simulink model "launch_gate_exp"  (R2022b)
settings: Solver=FixedStepDiscrete  StartTime=0.0  StopTime=5  FixedStep=0.001  RelTol=1e-3
InitFcn:
  | if ~exist('P','var') || ~isfield(P,'gate_version'), P=gate_params(launch_tcs_params()); end
model workspace (MAT data in the model file):
  w_2 : Simulink.Parameter (value not decoded)
undefined symbols (not defined in the file): A, a, B, b, C, D, DiscIntNeverNeededParam, Iz, K, k1, K1, k2, K2, L1, L2, m, magnitude, Phi, Sample_time, Steer_Ratio
libraries: simulink x26, slpidlib x13, Solver_SF x1, dsparch4 x1
(part 7 of 7)

== matlab function launch_gate_exp/PID_Controller//直线循迹/MATLAB Function2 ==
  data: st input; flag_ctrl output; flag_cnt output; yaw input; throttle input; yaw_ref output
function [flag_ctrl, flag_cnt, yaw_ref] = StraightModeDetector(st, yaw, throttle)

%% 实车调试版本
% 所有 persistent 变量必须为 single 以满足实车要求 
persistent ctrl_cnt yaw_sum yaw_time yaw_ref_int yaw_f
if isempty(ctrl_cnt)
    ctrl_cnt    = single(0);
    yaw_sum     = single(0);
    yaw_time    = single(0);
    yaw_ref_int = single(0);
    yaw_f       = single(0);
end

%% === 参数 ===
st_lim_enter = single(1);     % 进入判定阈值 (deg)
st_lim_exit  = single(1.2);     % 退出判定（滞回）
thr_min      = single(1);       % 油门下限 (%)
thr_max      = single(50);      % 油门上限 (%)


T_ctrl   = single(3.0);         % 需要检测的直行时间 (s)
Ts       = single(0.02);        % sample time
num_ctrl = single(T_ctrl / Ts); % 循环次数

alpha = single(0.15);           % LPF 低通滤波器系数
flag_cnt = single(0);           % 累加计算目标航向使能

%% === Step 1: LPF 过滤 yaw ===
yaw_f = yaw_f + alpha * (yaw - yaw_f);

%% === Step 2: 判断是否满足直行条件 ===
cond_enter = (abs(st) < st_lim_enter) && (throttle > thr_min) && (throttle < thr_max);
cond_exit  = (abs(st) > st_lim_exit)  || (throttle <= thr_min) || (throttle >= thr_max);

%% === Step 3: 计数器逻辑 ===
if cond_enter
    ctrl_cnt = ctrl_cnt + 1;
else
    ctrl_cnt = single(0);
end

%% === Step 4: yaw 采样（累加）===
if cond_enter && (ctrl_cnt <= num_ctrl)
    yaw_sum  = yaw_sum  + yaw_f;
    yaw_time = yaw_time + 1;
    flag_cnt = single(1);
end

%% === Step 5: 进入直线控制模式的瞬间冻结 yaw_ref ===
% if ctrl_cnt == num_ctrl
%     yaw_ref_int = yaw_sum / yaw_time;
% end
if (ctrl_cnt >= num_ctrl) && (yaw_time > 0) && (yaw_ref_int == 0)
    yaw_ref_int = yaw_sum / yaw_time;
end

%% === Step 6: 若退出模式，则清空状态 ===
if cond_exit
    ctrl_cnt    = single(0);
    yaw_sum     = single(0);
    yaw_time    = single(0);
    yaw_ref_int = single(0);
end

%% === Step 7: 输出 ===
flag_ctrl = single(ctrl_cnt >= num_ctrl);
yaw_ref   = yaw_ref_int;

end

== matlab function launch_gate_exp/PID_Controller//直线循迹/指数加权移动平均 ==
  data: uk input; y output; is_biased input

function y = ExpMovAvg(uk, is_biased)
% 指数加权移动平均滤波器
% 输入:
%   uk      : 当前输入值
%   is_biased: 是否应用偏差修正 (1=是, 0=否)
% 输出:
%   y       : 指数加权移动平均值

% 持久变量保持状态 (在时间步之间保留值)
persistent shadow count first_time decay

% 初始化参数和状态
if isempty(first_time)
    % 初始化标志
    first_time = true;
    
    % 初始化状态值
    shadow = double(0);
    count = 0;
    
    % 设置衰减因子 (0.9是常用值，可根据需要修改)
    decay = 0.9;
end

% 主处理逻辑
if first_time
    % 第一次调用 - 初始化状态
    shadow = double(uk);
    count = 1;
    first_time = false;
    y = uk;  % 第一次返回当前值
else
    % 更新计数器
    count = count + 1;
    
    % 计算指数加权平均值
     a = decay * shadow + (1 - decay) * uk;
    shadow = double(a);
    
    if is_biased
        % 应用偏差修正 (1 - decay^count)
        bias_correction = 1 - decay^count;
         b = shadow / bias_correction;
        y = single(b);
    else
        % 返回原始加权平均值
        y = single(shadow);
    end
end
end

== matlab function launch_gate_exp/PID_Controller//直线循迹/模式判断 ==
  data: v input; st input; avg input; mode output
function mode  = stateflow(v,st,avg)

mode = 7; %常规模式

% 沥青路面判断
    if avg <= 2
        if v > 20
            if st>=8
                mode = 1; % 高速转向
            elseif st<=3
                mode = 2; % 高速直行
            end
        elseif v < 10
            if st>=5
                mode = 3; % 低速转向
            elseif st<5
                mode = 4; % 低速直行
            end
        end
    % 土地路面判断
    elseif avg >= 3
        if v >= 10
            mode = 5; % 土地快速
        elseif v < 10
            mode = 6; % 土地低速
        end
    end
end

== matlab function launch_gate_exp/软土扭矩分配/滑移跟踪与扭矩生成 ==
  data: kappa input; nominal_torques_n_m output; kappa_valid input; input_gains input; adaptive_targets input; base_torques_n_m input; wheel_limits_n_m input; slip_errors output
function [nominal_torques_n_m, slip_errors] = MF_SlipTrackingNominalTorque(kappa, kappa_valid, input_gains, adaptive_targets, base_torques_n_m, wheel_limits_n_m)

% 滑移跟踪与名义扭矩生成模块
%
% 根据四轮实际滑移率与四轮目标滑移率之间的误差，生成名义轮端扭矩。
%
% 名义扭矩不是最终输出扭矩，后续还需要经过 CBF-QP 模块进行安全约束和协调分配。

%% 输入整理

kappa_vec = row4_local(kappa);
valid_vec = row4_local(kappa_valid);
gain_vec = row4_local(input_gains);
target_vec = row4_local(adaptive_targets);
base_vec = row4_local(base_torques_n_m);
limit_vec = row4_local(wheel_limits_n_m);

%% 控制参数

% 滑移率误差到扭矩修正的比例增益。
slip_tracking_gain = 20500.0;

% 单轮扭矩修正量限幅。
torque_delta_limit = 2600.0;

%% 四轮名义扭矩计算

nominal_torques_n_m = zeros(1, 4);
slip_errors = zeros(1, 4);

for index = 1:4

    wheel_limit = max(0.0, limit_vec(index));
    base_torque = clamp_local(base_vec(index), 0.0, wheel_limit);

    if valid_vec(index) > 0.5 && isfinite(kappa_vec(index)) && isfinite(target_vec(index)) && isfinite(gain_vec(index))

        % 四轮独立滑移率跟踪误差。
        slip_errors(index) = kappa_vec(index) - target_vec(index);

        % 滑移率反馈扭矩修正。
        % 若实际滑移率大于目标，误差为正，扭矩修正为负，降低驱动扭矩；
        % 若实际滑移率小于目标，误差为负，扭矩修正为正，提高驱动扭矩。
        torque_delta = -slip_tracking_gain * slip_errors(index);

        % 扭矩修正限幅。
        torque_delta = clamp_local(torque_delta, -torque_delta_limit, torque_delta_limit);

        nominal = base_torque + torque_delta;

    else

        % 滑移率或输入增益无效时，不做滑移反馈修正，保持基线扭矩。
        slip_errors(index) = 0.0;
        nominal = base_torque;
    end

    % 名义扭矩满足物理轮端限幅。
    nominal_torques_n_m(index) = clamp_local(nominal, 0.0, wheel_limit);
end

end


function output = row4_local(values)

% 将输入信号整理为 1×4 行向量。

input_values = double(values);
output = zeros(1, 4);

for index = 1:4
    output(index) = input_values(index);
end

end


function value = clamp_local(value_in, lower, upper)

% 数值限幅函数。

value = min(max(double(value_in), double(lower)), double(upper));

end

== matlab function launch_gate_exp/软土扭矩分配/CBF-QP扭矩分配 ==
  data: dt_s input; selected_torques_n_m output; kappa input; dot_kappa input; kappa_valid input; input_gains input; previous_applied_torques_n_m input; nominal_torques_n_m input; base_torques_n_m input; wheel_limits_n_m input; front_steers_rad input; total_torque_n_m input; control_mz_n_m input; cbf_torque_upper_bounds output; cbf_active output; qp_status output; qp_objective output; disturbance_state_out output; disturbance_margins output
function [selected_torques_n_m, cbf_torque_upper_bounds, cbf_active, qp_status, qp_objective, disturbance_state_out, disturbance_margins] = MF_CBF_QP_TorqueAllocator(dt_s, kappa, dot_kappa, kappa_valid, input_gains, previous_applied_torques_n_m, nominal_torques_n_m, base_torques_n_m, wheel_limits_n_m, front_steers_rad, total_torque_n_m, control_mz_n_m)

% CBF-QP 安全扭矩分配模块
%
% 本模块完成：
% 1）滑移率动力学扰动估计；
% 2）CBF滑移安全扭矩上界计算；
% 3）考虑前轮转角的横摆力矩系数计算；
% 4）四轮扭矩QP优化分配。

persistent disturbance_state

if isempty(disturbance_state)
    disturbance_state = zeros(1, 4);
end

%% 输入整理

dt = max(double(dt_s), 0.0);

kappa_vec = row4_local(kappa);
dot_kappa_vec = row4_local(dot_kappa);
valid_vec = row4_local(kappa_valid);
gain_vec = row4_local(input_gains);
applied_vec = row4_local(previous_applied_torques_n_m);
nominal_vec = row4_local(nominal_torques_n_m);
base_vec = row4_local(base_torques_n_m);
limit_vec = row4_local(wheel_limits_n_m);

total_target = double(total_torque_n_m);
yaw_target = double(control_mz_n_m);

steer_input = double(front_steers_rad);

if numel(steer_input) >= 2
    delta_l = steer_input(1);
    delta_r = steer_input(2);
else
    delta_l = steer_input(1);
    delta_r = steer_input(1);
end

%% 轮端限幅整理

wheel_limits = zeros(1, 4);
base_torques = zeros(1, 4);
nominal_torques = zeros(1, 4);

for index = 1:4

    wheel_limits(index) = max(0.0, limit_vec(index));

    base_torques(index) = clamp_local(base_vec(index), 0.0, wheel_limits(index));

    nominal_torques(index) = clamp_local(nominal_vec(index), 0.0, wheel_limits(index));
end

%% 一、等效扰动估计

% 滑移率动力学：
% dot(kappa_i) = g_i * T_i + d_i
%
% 等效扰动估计：
% d_i = dot(kappa_i) - g_i * T_i

disturbance_margins = zeros(1, 4);
alpha_disturbance = first_order_alpha_local(dt, 0.15);

for index = 1:4

    gain = gain_vec(index);

    if valid_vec(index) > 0.5 && isfinite(gain)

        raw_estimate = dot_kappa_vec(index) - gain * applied_vec(index);

        disturbance_state(index) = disturbance_state(index) + ...
            alpha_disturbance * (raw_estimate - disturbance_state(index));

        residual = raw_estimate - disturbance_state(index);

    else

        residual = 0.0;
    end

    % 扰动估计不确定性裕度。
    disturbance_margins(index) = clamp_local(0.05 + 0.05 * abs(residual), 0.05, 5.0);
end

disturbance_state_out = disturbance_state;

%% 二、CBF滑移安全扭矩上界计算

% 安全函数：
% h_i = kappa_max - kappa_i
%
% CBF条件：
% dot(h_i) + gamma*h_i >= 0
%
% 由 dot(kappa_i) = g_i*T_i + d_i 可得：
% g_i*T_i + d_i + margin_i <= gamma*(kappa_max - kappa_i)
%
% 因此：
% T_i <= [gamma*(kappa_max-kappa_i) - d_i - margin_i] / g_i

kappa_max = 0.25;
cbf_gamma = 15.0;

cbf_torque_upper_bounds = zeros(1, 4);
cbf_active = zeros(1, 4);

for index = 1:4

    gain = gain_vec(index);

    if valid_vec(index) > 0.5 && isfinite(gain) && isfinite(kappa_vec(index))

        upper = (cbf_gamma * (kappa_max - kappa_vec(index)) ...
            - disturbance_state(index) ...
            - disturbance_margins(index)) / gain;

        if ~isfinite(upper)
            upper = wheel_limits(index);
        end

        upper = clamp_local(upper, 0.0, wheel_limits(index));

    else

        upper = wheel_limits(index);
    end

    cbf_torque_upper_bounds(index) = upper;

    % 若CBF上界低于基线扭矩，说明安全约束实际参与限幅。
    if upper < base_torques(index) - 1.0e-6
        cbf_active(index) = 1.0;
    end
end

%% 三、考虑前轮转角的横摆力矩映射系数

% 车辆几何参数。
lf = 2.043;
lr = 1.362;

track_front = 2.39;
track_rear = 2.33;

radius_front = 0.834;
radius_rear = 0.94;

% 当前QP只考虑轮端纵向驱动力产生的横摆力矩。
% 对前轮，驱动力方向随转角变化：
% F_x_body = F_i*cos(delta_i)
% F_y_body = F_i*sin(delta_i)
%
% 横摆力矩：
% M_z_i = x_i*F_y_body - y_i*F_x_body
%
% 因为 F_i = T_i/r_i，所以：
% yaw_coeff_i = (x_i*sin(delta_i) - y_i*cos(delta_i)) / r_i

yaw_coefficients = zeros(1, 4);

% 左前轮：x = lf, y = +track_front/2。
yaw_coefficients(1) = (lf * sin(delta_l) - 0.5 * track_front * cos(delta_l)) / radius_front;

% 右前轮：x = lf, y = -track_front/2。
yaw_coefficients(2) = (lf * sin(delta_r) + 0.5 * track_front * cos(delta_r)) / radius_front;

% 左后轮：x = -lr, y = +track_rear/2, delta = 0。
% 因为 sin(0)=0，所以 lr 项不直接进入纵向力横摆力矩。
yaw_coefficients(3) = -0.5 * track_rear / radius_rear;

% 右后轮：x = -lr, y = -track_rear/2, delta = 0。
yaw_coefficients(4) = 0.5 * track_rear / radius_rear;

%% 四、QP四轮扭矩优化分配

lower_bounds = zeros(1, 4);

[qp_torques, qp_status, qp_objective] = solve_torque_qp_local( ...
    nominal_torques, ...
    total_target, ...
    yaw_target, ...
    lower_bounds, ...
    cbf_torque_upper_bounds, ...
    yaw_coefficients);

%% 五、QP失败时安全降级

if qp_status > 0.5

    selected_torques_n_m = qp_torques;

else

    selected_torques_n_m = zeros(1, 4);

    for index = 1:4
        selected_torques_n_m(index) = clamp_local(base_torques(index), 0.0, cbf_torque_upper_bounds(index));
    end
end

end


function [solution, status, objective] = solve_torque_qp_local(nominal, total_target, yaw_target, lower, upper, yaw)

% 四轮扭矩边界约束QP求解器
%
% 决策变量：
% T = [T1, T2, T3, T4]
%
% 目标函数：
% J = 0.5*w_nominal*sum((T_i - T_nom_i)^2)
%   + 0.5*w_total*(sum(T_i) - T_total_ref)^2
%   + 0.5*w_yaw*(yaw*T' - Mz_ref)^2
%   + regularization*sum(T_i^2)
%
% 约束：
% lower_i <= T_i <= upper_i
%
% 由于只有4个决策变量，这里采用主动集枚举方法，
% 每个变量枚举为下界、自由、上界三种状态。

status = -1.0;
objective = NaN;
solution = zeros(1, 4);

%% 可行性预检查

for index = 1:4
    if upper(index) < lower(index) || ~isfinite(upper(index)) || ~isfinite(lower(index))
        return;
    end
end

%% 权重参数

weight_nominal = 1.0;
weight_total = 1.12;
weight_yaw = 0.02;
regularization = 1.0e-6;

%% 构造二次型矩阵和线性项

H = zeros(4, 4);
linear = zeros(1, 4);

for row = 1:4

    for col = 1:4

        % 总扭矩项对 Hessian 的贡献。
        % 横摆力矩项对 Hessian 的贡献。
        H(row, col) = H(row, col) + weight_total + weight_yaw * yaw(row) * yaw(col);
    end

    % 名义扭矩跟踪项和正则化项。
    H(row, row) = H(row, row) + weight_nominal + 2.0 * regularization;

    % 线性项。
    linear(row) = linear(row) ...
        - weight_nominal * nominal(row) ...
        - weight_total * total_target ...
        - weight_yaw * yaw_target * yaw(row);
end

%% 主动集枚举

best_objective = Inf;

% -1：固定在下界；
%  0：自由变量；
%  1：固定在上界。
states = [-1.0, 0.0, 1.0];

for i1 = 1:3
    for i2 = 1:3
        for i3 = 1:3
            for i4 = 1:3

                activity = [states(i1), states(i2), states(i3), states(i4)];

                candidate = zeros(1, 4);
                free_indices = zeros(1, 4);
                nfree = 0;

                %% 设置固定变量并记录自由变量

                for index = 1:4

                    if activity(index) < -0.5

                        candidate(index) = lower(index);

                    elseif activity(index) > 0.5

                        candidate(index) = upper(index);

                    else

                        nfree = nfree + 1;
                        free_indices(nfree) = index;
                    end
                end

                %% 求解自由变量

                if nfree > 0

                    A = zeros(4, 4);
                    b = zeros(1, 4);

                    for rr = 1:nfree

                        row = free_indices(rr);
                        fixed_contribution = 0.0;

                        for col = 1:4
                            if activity(col) ~= 0.0
                                fixed_contribution = fixed_contribution + H(row, col) * candidate(col);
                            end
                        end

                        b(rr) = -linear(row) - fixed_contribution;

                        for cc = 1:nfree
                            A(rr, cc) = H(row, free_indices(cc));
                        end
                    end

                    [free_solution, ok] = solve_linear_system4_local(A, b, nfree);

                    if ok <= 0.5
                        continue;
                    end

                    for rr = 1:nfree
                        candidate(free_indices(rr)) = free_solution(rr);
                    end
                end

                %% 可行性检查

                feasible = 1.0;

                for index = 1:4

                    if candidate(index) < lower(index) - 1.0e-7 || ...
                            candidate(index) > upper(index) + 1.0e-7 || ...
                            ~isfinite(candidate(index))

                        feasible = 0.0;
                    end

                    candidate(index) = clamp_local(candidate(index), lower(index), upper(index));
                end

                if feasible <= 0.5
                    continue;
                end

                %% 计算目标函数

                obj = quadratic_objective_local(candidate, H, linear);

                if obj < best_objective

                    best_objective = obj;
                    solution = candidate;
                    status = 1.0;
                    objective = obj;
                end
            end
        end
    end
end

end


function [x, ok] = solve_linear_system4_local(A, b, n)

% 求解最多4维线性方程组 A*x=b。
% 采用带部分主元选择的高斯消元法。

x = zeros(1, 4);
ok = 1.0;

if n == 0
    return;
end

aug = zeros(4, 5);

for row = 1:n

    for col = 1:n
        aug(row, col) = A(row, col);
    end

    aug(row, n + 1) = b(row);
end

%% 前向消元

for col = 1:n

    pivot_row = col;
    pivot_abs = abs(aug(col, col));

    for row = col:n
        if abs(aug(row, col)) > pivot_abs
            pivot_abs = abs(aug(row, col));
            pivot_row = row;
        end
    end

    if pivot_abs <= 1.0e-12 || ~isfinite(pivot_abs)
        ok = 0.0;
        return;
    end

    if pivot_row ~= col

        temp = aug(col, :);
        aug(col, :) = aug(pivot_row, :);
        aug(pivot_row, :) = temp;
    end

    for row = col + 1:n

        factor = aug(row, col) / aug(col, col);

        if factor ~= 0.0

            for entry = col:n + 1
                aug(row, entry) = aug(row, entry) - factor * aug(col, entry);
            end
        end
    end
end

%% 回代

for row = n:-1:1

    residual = aug(row, n + 1);

    for col = row + 1:n
        residual = residual - aug(row, col) * x(col);
    end

    pivot = aug(row, row);

    if abs(pivot) <= 1.0e-12
        ok = 0.0;
        return;
    end

    x(row) = residual / pivot;

    if ~isfinite(x(row))
        ok = 0.0;
        return;
    end
end

end


function value = quadratic_objective_local(torques, H, linear)

% QP目标函数：
% J = 0.5*T*H*T' + linear*T'

value = 0.0;

for row = 1:4

    for col = 1:4
        value = value + 0.5 * torques(row) * H(row, col) * torques(col);
    end

    value = value + linear(row) * torques(row);
end

end


function output = row4_local(values)

% 将输入信号整理为 1×4 行向量。

input_values = double(values);
output = zeros(1, 4);

for index = 1:4
    output(index) = input_values(index);
end

end


function alpha = first_order_alpha_local(dt, time_constant_s)

% 一阶低通滤波系数。

if dt <= 0.0 || time_constant_s <= 0.0
    alpha = 1.0;
else
    alpha = dt / (time_constant_s + dt);
end

end


function value = clamp_local(value_in, lower, upper)

% 数值限幅函数。

value = min(max(double(value_in), double(lower)), double(upper));

end

== matlab function launch_gate_exp/软土扭矩分配/牵引效率评价计算 ==
  data: dt_s input; eta_wg_E output; drawbar_power_w input; wheel_power_w input; E_wg output; E_w output; drawbar_force input
function [eta_wg_E, E_wg, E_w] = MF_EnergyWeightedTractionEfficiency(dt_s, drawbar_power_w, wheel_power_w, drawbar_force)

persistent E_wg_state E_w_state

if isempty(E_wg_state)
    E_wg_state = 0.0;
    E_w_state = 0.0;
end

dt = max(double(dt_s), 0.0);

epsilon_E = 1.0;   % 防止低能量窗口除零，可根据功率量级调整

%window_enable = wheel_power_w > 100 && drawbar_force > 10;
window_enable = 1;

if double(window_enable) > 0.5
    E_wg_state = E_wg_state + max(0.0, double(drawbar_power_w)) * dt;
    E_w_state = E_w_state + max(0.0, double(wheel_power_w)) * dt;
end

eta_wg_E = E_wg_state / (E_w_state + epsilon_E);

E_wg = E_wg_state;
E_w = E_w_state;

end

== matlab function launch_gate_exp/Implement_Load/Load_Model ==
  data: t input; D output; vg input; s input; D0 parameter; B parameter; C parameter; LoadMode parameter; LoadStart parameter; UseDistance parameter; StartDistance parameter; D_unlimited output; u_imp output; vg_record output; RampTime parameter; DMax parameter
function [D,D_unlimited,u_imp,vg_record] = Load_Model(t,vg,s,D0,B,C,LoadMode,LoadStart,UseDistance,StartDistance,RampTime, DMax)
%#codegen
% Equivalent longitudinal resistance, N; NOT identified ASABE coefficients.
% Mode 0: constant interface diagnostic; mode 1: parametric subsoiler assumption.
vg_record=0;D_unlimited=0;u_imp=0;D=0;
if ~isfinite(t)||~isfinite(vg)||~isfinite(D0)||~isfinite(B)||~isfinite(C)||~isfinite(DMax)||DMax<0
 return;
end
vg_record=vg;v=max(vg,0);
steady=D0;
if LoadMode>0.5,steady=D0+B*v+C*v*v;end
if ~isfinite(steady),return;end
if ~isfinite(LoadStart)||~isfinite(RampTime),return;end
if UseDistance>0.5
 if ~isfinite(s)||~isfinite(StartDistance)||s<StartDistance,return;end
end
u_imp=min(max((t-LoadStart)/max(RampTime,1e-3),0),1);
D_unlimited=u_imp*max(steady,0);
D=min(D_unlimited,DMax);
end

== matlab function launch_gate_exp/Common motor capability ==
  data: raw input; T output; cap input
function T = common_cap(raw,cap)
%#codegen
T=zeros(4,1);
for i=1:4
 if isfinite(raw(i)) && isfinite(cap(i)) && cap(i)>=0
 T(i)=min(max(raw(i),0),cap(i));
 end
end
end

== matlab function launch_gate_exp/驱动防滑模块/起步探测 ==
  data: v_ref output size=[4 1]; dv output size=[4 1]; spin_on_raw output boolean size=[4 1]; spin_clear_raw output boolean size=[4 1]; no_move_raw output boolean; w input size=[4 1]; vx input; vy input; ax input; r input; delta input size=[4 1]; speed_src_valid input; T_actual input size=[4 1]; T_max input size=[4 1]; reset input; move_ok output boolean; speed_on_raw output boolean; speed_off_raw output boolean; consistency_ok output boolean; source_immediate_bad output boolean; drive_active output boolean; diag_motion output size=[4 1]; P parameter; dv_ctrl output; dv_rate_ctrl output; fast_worsening output; active_out output
function [v_ref, dv, spin_on_raw, spin_clear_raw, no_move_raw, move_ok, ...
          speed_on_raw, speed_off_raw, consistency_ok, ...
          source_immediate_bad, drive_active, diag_motion, ...
          dv_ctrl, dv_rate_ctrl, fast_worsening, active_out] = ...
    LaunchTCS_Motion(w, vx, vy, ax, r, delta, speed_src_valid, ...
                     T_actual, T_max, reset, P)
%#codegen
% 前级：只计算运动量和瞬时判据，不做计时、不锁存、不决定 stage。
% 四轮顺序 [FL;FR;RL;RR]。

persistent initialized w_f vx_f vy_f ax_f r_f vx_prev dv_prev dv_ctrl_f dv_ctrl_prev

if isempty(initialized)
    initialized = false;
    w_f = zeros(4,1); vx_f = 0; vy_f = 0; ax_f = 0; r_f = 0;
    vx_prev = 0; dv_prev = zeros(4,1);
    dv_ctrl_f = zeros(4,1); dv_ctrl_prev = zeros(4,1);
end

%% 1. 先统一定义所有局部变量（避免"未定义"报错）
w_s = zeros(4,1);
delta_s = zeros(4,1);
vx_s = 0; vy_s = 0; ax_s = 0; r_s = 0;
raw_ok = true;
vx_dot = 0;
v_ref = zeros(4,1);
dv = zeros(4,1);
wheel_speed = zeros(4,1);
dv_rate = zeros(4,1);
dv_ctrl = zeros(4,1);
dv_rate_ctrl = zeros(4,1);
active = zeros(4,1);

%% 2. 输入检查：异常值用上一拍滤波值顶替，并记录故障
for i = 1:4
    w_s(i) = w(i);
    delta_s(i) = delta(i);
    if isnan(w_s(i)) || isinf(w_s(i))
        w_s(i) = w_f(i); raw_ok = false;
    end
    if isnan(delta_s(i)) || isinf(delta_s(i))
        delta_s(i) = 0; raw_ok = false;
    end
end

vx_s = vx; vy_s = vy; ax_s = ax; r_s = r;
if isnan(vx_s) || isinf(vx_s), vx_s = vx_f; raw_ok = false; end
if isnan(vy_s) || isinf(vy_s), vy_s = vy_f; raw_ok = false; end
if isnan(ax_s) || isinf(ax_s), ax_s = ax_f; raw_ok = false; end
if isnan(r_s)  || isinf(r_s),  r_s  = r_f;  raw_ok = false; end

src_flag_ok = ~(isnan(speed_src_valid) || isinf(speed_src_valid));
src_val = speed_src_valid;
if ~src_flag_ok, src_val = 0; end

%% 3. 滤波与车速微分
do_init = (reset > 0.5) || ~initialized;
if do_init
    initialized = true;
    w_f = w_s; vx_f = vx_s; vy_f = vy_s; ax_f = ax_s; r_f = r_s;
    vx_prev = vx_f;
    dv_prev = zeros(4,1);
    dv_ctrl_f = zeros(4,1);
    dv_ctrl_prev = zeros(4,1);
else
    vx_prev = vx_f;
    w_f  = (1-P.alpha_w)  * w_f  + P.alpha_w  * w_s;
    vx_f = (1-P.alpha_v)  * vx_f + P.alpha_v  * vx_s;
    vy_f = (1-P.alpha_vy) * vy_f + P.alpha_vy * vy_s;
    ax_f = (1-P.alpha_a)  * ax_f + P.alpha_a  * ax_s;
    r_f  = (1-P.alpha_r)  * r_f  + P.alpha_r  * r_s;
end
vx_dot = (vx_f - vx_prev) / P.Ts;

%% 4. 四轮参考速度与轮端-车体速度差
for i = 1:4
    v_ref(i) = max(0, (vx_f - r_f*P.y(i))*cos(delta_s(i)) ...
                     + (vy_f + r_f*P.x(i))*sin(delta_s(i)));
    wheel_speed(i) = max(w_f(i), 0) * P.R(i);
    dv(i) = wheel_speed(i) - v_ref(i);
    if do_init
        dv_rate(i) = 0;
    else
        dv_rate(i) = (dv(i) - dv_prev(i)) / P.Ts;
    end
end

% Filtered, nonnegative dv is used only by control and Stateflow判据.
% The raw signed dv output remains unchanged for diagnostics.
alpha_dv_ctrl = P.Ts / (max(P.tau_dv_ctrl,1.0e-6) + P.Ts);
if do_init
    dv_ctrl_f = dv;
    dv_ctrl_prev = dv_ctrl_f;
    dv_ctrl = max(dv_ctrl_f,0);
    dv_rate_ctrl = zeros(4,1);
else
    dv_ctrl_prev = dv_ctrl_f;
    dv_ctrl_f = dv_ctrl_f + alpha_dv_ctrl * (dv - dv_ctrl_f);
    dv_ctrl = max(dv_ctrl_f,0);
    dv_rate_ctrl = (dv_ctrl - max(dv_ctrl_prev,0)) / P.Ts;
end

%% 5. 信号健康与有效驱动
plausible = (vx_f >= P.vx_min) && (vx_f <= P.vx_max);
src_ok = (src_val > 0.5) && src_flag_ok;
actual_ok = true;

for i = 1:4
    cap_valid = ~(isnan(T_max(i)) || isinf(T_max(i))) && ...
                (T_max(i) >= P.TcapFloor(i));
    act_valid = ~(isnan(T_actual(i)) || isinf(T_actual(i)));
    if ~act_valid, actual_ok = false; end
    if cap_valid && act_valid
        active(i) = double(T_actual(i) >= P.applied_active_frac * T_max(i));
    end
end

drive_active = any(active > 0.5);
source_immediate_bad = (~raw_ok) || (~src_ok) || (~plausible) || ...
                       (~actual_ok);
consistency_ok = (~source_immediate_bad) && ...
                 (abs(vx_dot - ax_f) <= P.a_cons_max);

%% 6. 四轮空转瞬时条件
spin_on_raw = false(4,1);
spin_clear_raw = false(4,1);
fast_worsening = false(4,1);
active_out = active > 0.5;
for i = 1:4
    spin_on_raw(i) = (~source_immediate_bad) && ...
        (dv_ctrl(i) > P.dv_spin_on) && ...
        (wheel_speed(i) > P.v_wheel_min) && ...
        (active(i) > 0.5);
    % Sustained-slip evidence does not disappear when growth slows.
    fast_worsening(i) = (~source_immediate_bad) && (active(i)>0.5) && ...
        (dv_ctrl(i)>P.dv_fast_on) && (dv_rate_ctrl(i)>P.dv_growth_on);
    spin_clear_raw(i) = (~source_immediate_bad) && (dv_ctrl(i) < P.dv_spin_off);
end

%% 7. 未起动与车速切换瞬时条件
no_move_raw = (~source_immediate_bad) && drive_active && ...
              (vx_f < P.v_move_on) && (ax_f < P.a_response);
move_ok = (~source_immediate_bad) && ...
          ((vx_f >= P.v_move_on) || (ax_f >= P.a_response));
speed_on_raw = (~source_immediate_bad) && consistency_ok && ...
               (vx_f >= P.v_valid_on);
speed_off_raw = source_immediate_bad || (vx_f < P.v_valid_off);

%% 8. 观察量与历史更新
diag_motion = [vx_f; ax_f; vx_dot; max(dv)];
dv_prev = dv;

end

== matlab function launch_gate_exp/驱动防滑模块/起步扭矩控制 ==
  data: stage input uint8; T_pref output size=[4 1]; spin_mask input boolean size=[4 1]; dv_ctrl input size=[4 1]; T_base input size=[4 1]; T_max input size=[4 1]; reset input; fast_worsening input size=[4 1]; prewarn input boolean size=[4 1]; warn_age input double size=[4 1]; T_actual_prev input double size=[4 1]; vx_raw input double size=[1 1]; source_bad input boolean size=[1 1]; T_lim_out output size=[4 1]; T_cmd output size=[4 1]; diag_torque output size=[4 1]; P parameter; T_pref_open output; I_dv_out output; cap_out output; T_target output; T_slip_lim output; slip_ratio_out output; slip_recovering output; cut_f_out output; gate_diag output double size=[72 1]
function [T_pref,T_lim_out,T_cmd,diag_torque,T_pref_open,I_dv_out,cap_out,T_target,T_slip_lim,slip_ratio_out,slip_recovering,cut_f_out,gate_diag] = ...
 LaunchTCS_Torque(stage,spin_mask,dv_ctrl,T_base,T_max,reset,fast_worsening,prewarn,warn_age,T_actual_prev,vx_raw,source_bad,P)
%#codegen
% Stateflow owns warning/confirmed events. This block only shapes actuator bounds.
% No P/I/fast-P correction and no cut_f persistent state exists.
persistent initialized envelope bound bound_target anchor previous_warning previous_spin previous_cmd multi_bound multi_anchor multi_previous exit_timer handed_off
if isempty(initialized)
 initialized=true;envelope=zeros(4,1);bound=ones(4,1)*1e12;bound_target=ones(4,1)*1e12;anchor=zeros(4,1);
 previous_warning=false(4,1);previous_spin=false(4,1);previous_cmd=zeros(4,1);
 multi_bound=1e12;multi_anchor=0;multi_previous=false;exit_timer=0;handed_off=false;
end
cap=zeros(4,1);base=zeros(4,1);applied=zeros(4,1);rated=max(P.TcapDefault,1);
input_bad=source_bad || ~isfinite(vx_raw);
for i=1:4
 if isfinite(T_max(i)) && T_max(i)>=0,cap(i)=T_max(i);else,input_bad=true;end
 if isfinite(T_base(i)),base(i)=max(T_base(i),0);else,input_bad=true;end
 if isfinite(T_actual_prev(i)),applied(i)=max(T_actual_prev(i),0);else,input_bad=true;end
 if ~isfinite(dv_ctrl(i)),input_bad=true;end
end
T_pref=zeros(4,1);T_lim_out=cap;T_cmd=zeros(4,1);diag_torque=zeros(4,1);
T_pref_open=zeros(4,1);I_dv_out=zeros(4,1);cap_out=cap;T_target=zeros(4,1);
T_slip_lim=cap;slip_ratio_out=ones(4,1);slip_recovering=false(4,1);cut_f_out=zeros(4,1);
gate_diag=zeros(72,1);
if reset>0.5 || stage==uint8(255)
 envelope=zeros(4,1);bound=ones(4,1)*1e12;bound_target=ones(4,1)*1e12;anchor=zeros(4,1);previous_cmd=zeros(4,1);
 previous_warning=false(4,1);previous_spin=false(4,1);multi_bound=1e12;multi_anchor=0;
 multi_previous=false;exit_timer=0;handed_off=false;return;
end
protect=input_bad || stage==uint8(6);
if vx_raw>=P.gate_exit_speed && ~protect,exit_timer=min(P.gate_exit_hold,exit_timer+P.Ts);else,exit_timer=0;end
if exit_timer>=P.gate_exit_hold,handed_off=true;end
% Re-enter launch supervision only after an actual return to near standstill.
if handed_off && vx_raw<.1 && stage<=uint8(1),handed_off=false;exit_timer=0;end
nconfirmed=sum(double(spin_mask));multi=(nconfirmed>=2)&&~handed_off;
for i=1:4
 warning=prewarn(i)&&~handed_off;confirmed=spin_mask(i)&&~handed_off;
 warning_rise=warning && ~previous_warning(i);
 confirmed_rise=confirmed && ~previous_spin(i);
 if warning_rise || confirmed_rise
  % Capture already applied torque once; changes of motor cap do not update anchor.
  anchor(i)=max(applied(i),min(base(i),cap(i)));
 end
 if handed_off
  envelope(i)=max(envelope(i),applied(i));
  envelope(i)=min(base(i),envelope(i)+P.gate_handoff_rate*rated(i)*P.Ts);
  if bound(i)<base(i),bound(i)=min(base(i),bound(i)+P.gate_handoff_rate*rated(i)*P.Ts);end
 elseif confirmed
  if confirmed_rise
   bound_target(i)=max(P.gate_abs_floor,P.gate_spin_ratio*max(applied(i),0));
  end
  bound(i)=max(bound_target(i),bound(i)-P.gate_spin_cut_rate*rated(i)*P.Ts);
 elseif warning
  if warning_rise
   bound_target(i)=max(applied(i),P.gate_warn_ratio*anchor(i));
  end
  if warn_age(i)>=P.gate_escalate_delay && (fast_worsening(i) || dv_ctrl(i)>=P.dv_spin_on)
   bound(i)=max(bound_target(i),bound(i)-P.gate_warn_cut_rate*rated(i)*P.Ts);
  end
 else
  % Normal launch follows the common executable demand immediately; only
  % the shared command-rate limiter shapes the actuator trajectory.
  if stage==uint8(2)
   envelope(i)=min(base(i),max(envelope(i),applied(i))+P.gate_no_move_rate*rated(i)*P.Ts);
  else
   envelope(i)=min(base(i),cap(i));
  end
  bound_target(i)=min(base(i),cap(i));
  if bound(i)<bound_target(i),bound(i)=min(bound_target(i),bound(i)+P.gate_recover_rate*rated(i)*P.Ts);end
 end
 % Demand reductions may lower the command but do not invent extra safety memory.
 T_pref_open(i)=min(base(i),max(envelope(i),0));
 T_pref(i)=T_pref_open(i);T_slip_lim(i)=min(base(i),max(bound(i),0));
 T_lim_out(i)=min(cap(i),T_slip_lim(i));
 if protect,T_lim_out(i)=min(T_lim_out(i),P.q_protect*cap(i));end
 T_target(i)=min(T_pref(i),T_lim_out(i));
 previous_warning(i)=warning;previous_spin(i)=confirmed;
end
% One total bound is intersected with wheel bounds; penalties are not multiplied.
sum_target=sum(T_target);
if multi && ~multi_previous,multi_anchor=sum(applied);multi_bound=multi_anchor;end
if multi
 multi_bound=max(P.gate_multi_ratio*multi_anchor,multi_bound-P.gate_multi_cut_rate*sum(rated)*P.Ts);
elseif multi_bound<sum(base)
 multi_bound=min(sum(base),multi_bound+P.gate_multi_recover_rate*sum(rated)*P.Ts);
end
multi_previous=multi;
multi_scale=1;if sum_target>multi_bound && sum_target>0,multi_scale=max(multi_bound,0)/sum_target;end
transfer=zeros(4,1);
% Optional candidate: only healthy, unconfirmed, unwarned receivers with headroom.
if P.gate_redistribute>0 && ~protect && ~handed_off
 lost=sum(max(base-T_target,0));room=zeros(4,1);
 for i=1:4
  if ~prewarn(i)&&~spin_mask(i),room(i)=max(0,min(cap(i),envelope(i))-T_target(i));end
 end
 if sum(room)>0
  transfer=room/sum(room)*min(P.gate_redistribute*lost,sum(room));
  T_target=T_target+transfer;
 end
end
rate_cmd=zeros(4,1);hard_lim=zeros(4,1);override=zeros(4,1);
for i=1:4
 % The per-wheel hard limit is never raised to preserve a rate limit.
 hard_lim(i)=min(cap(i),min(base(i),max(T_lim_out(i),0)));
 if protect,hard_lim(i)=min(hard_lim(i),P.q_protect*cap(i));end
 T_lim_out(i)=hard_lim(i);
 target=min(max(T_target(i),0),hard_lim(i));
 prev=previous_cmd(i);
 if target>=prev,rate_cmd(i)=min(target,prev+P.gate_cmd_rise_rate*rated(i)*P.Ts);
 else,rate_cmd(i)=max(target,prev-P.gate_cmd_fall_rate*rated(i)*P.Ts);end
 rate_cmd(i)=min(max(rate_cmd(i),0),1e12);
end
% Project the rate-limited command onto the vehicle-level safety bound.
% This safety override is allowed to exceed the normal fall-rate and is
% recorded in gate_diag rather than hidden by increasing T_lim_out.
if multi && sum(rate_cmd)>multi_bound && sum(rate_cmd)>0
 safety_scale=max(multi_bound,0)/sum(rate_cmd);
else
 safety_scale=1;
end
for i=1:4
 T_cmd(i)=min(rate_cmd(i)*safety_scale,hard_lim(i));
 override(i)=max(rate_cmd(i)-T_cmd(i),0);
 slip_ratio_out(i)=min(max(bound(i)/max(base(i),1),0),1);
 slip_recovering(i)=~prewarn(i)&&~spin_mask(i)&&bound(i)<base(i);
 reason=0;
 if envelope(i)<base(i)-1,reason=1;end
 if prewarn(i)&&bound(i)<min(base(i),envelope(i))-1,reason=2;end
 if spin_mask(i)&&bound(i)<min(base(i),envelope(i))-1,reason=3;end
 if multi_scale<1,reason=4;end
 if cap(i)<min(base(i),min(envelope(i),bound(i)))-1,reason=5;end
 if abs(T_cmd(i)-target)>1,reason=6;end
 if protect,reason=8;end
 gate_diag(i)=envelope(i);gate_diag(4+i)=bound(i);gate_diag(8+i)=anchor(i);
 gate_diag(12+i)=double(prewarn(i));gate_diag(16+i)=double(spin_mask(i));
 gate_diag(20+i)=double(envelope(i)<min(base(i),cap(i))-1);
 gate_diag(24+i)=double(bound(i)<min(base(i),min(envelope(i),cap(i)))-1);
 gate_diag(28+i)=double(cap(i)<min(base(i),min(envelope(i),bound(i)))-1);
 gate_diag(32+i)=double(multi_scale<1);gate_diag(36+i)=reason;
 gate_diag(40+i)=double(handed_off);gate_diag(44+i)=transfer(i);
 gate_diag(48+i)=double(protect);gate_diag(52+i)=target;
 gate_diag(56+i)=double(slip_recovering(i));gate_diag(60+i)=multi_bound;
 gate_diag(64+i)=double(override(i)>1e-9);gate_diag(68+i)=override(i);
end
previous_cmd=T_cmd;diag_torque=[min(sum(envelope)/max(sum(base),1),1);multi_scale;nconfirmed;double(stage)];
end

== stateflow chart launch_gate_exp/驱动防滑模块/launch_state ==
  settings: updateMethod=DISCRETE  sampleTime=0.001
  state MONITOR [parallel]
    entry:
    spin_on_t=zeros(4,1); spin_clear_t=zeros(4,1); spin_mask=false(4,1); nspin=0; no_move_t=0;
    no_move_confirmed=false; speed_on_t=0; speed_off_t=0; speed_valid=false; cons_bad_t=0;
    source_bad=false; desired_stage=uint8(255);
    prewarn=false(4,1);warn_armed=true(4,1);warn_age=zeros(4,1);warn_on_t=zeros(4,1);warn_clear_t=zeros(4,1);warn_early_t=zeros(4,1);
    during:
    if enable<=0.5 || reset>0.5
    spin_on_t=zeros(4,1); spin_clear_t=zeros(4,1); spin_mask=false(4,1); nspin=0; no_move_t=0;
    no_move_confirmed=false; speed_on_t=0; speed_off_t=0; speed_valid=false; cons_bad_t=0;
    prewarn=false(4,1);warn_armed=true(4,1);warn_age=zeros(4,1);warn_on_t=zeros(4,1);warn_clear_t=zeros(4,1);warn_early_t=zeros(4,1);
    source_bad=false; if enable<=0.5, desired_stage=uint8(255); else, desired_stage=uint8(0);
    end
    else
    % Establish current-sample validity before warning supervision. A bad
    % source cancels warning immediately; the stage logic below still takes
    % source_bad to PROTECT without waiting for warning timers.
    if source_immediate_bad || ~consistency_ok
    cons_bad_t=min(P.t_cons_bad,cons_bad_t+P.Ts);
    else
    cons_bad_t=max(0,cons_bad_t-P.Ts);
    end
    source_bad=source_immediate_bad || cons_bad_t>=P.t_cons_bad;
    if source_bad
    prewarn=false(4,1); warn_armed=false(4,1); warn_age=zeros(4,1);
    warn_on_t=zeros(4,1); warn_clear_t=zeros(4,1); warn_early_t=zeros(4,1);
    else
    for i=1:4
    if ~prewarn(i) && ~spin_mask(i) && dv_warning(i)<P.gate_warn_off
    warn_armed(i)=true;
    end
    end
    end
    for i=1:4
    if spin_on_raw(i), spin_on_t(i)=min(P.t_spin_on,spin_on_t(i)+P.Ts); spin_clear_t(i)=0;
    else, spin_on_t(i)=max(0,spin_on_t(i)-P.Ts); if spin_clear_raw(i), spin_clear_t(i)=min(P.t_spin_clear,spin_clear_t(i)+P.Ts);
    else, spin_clear_t(i)=0;
    end, end
    if spin_on_t(i)>=P.t_spin_on, spin_mask(i)=true; end
    if spin_clear_t(i)>=P.t_spin_clear, spin_mask(i)=false; end
    end
    % Event supervision only: warning does not mask sustained spin evidence.
    for i=1:4
    if dv_warning(i)>=P.gate_warn_on
    warn_on_t(i)=min(P.gate_warn_delay,warn_on_t(i)+P.Ts);
    else
    warn_on_t(i)=0;
    end
    if dv_warning(i)>=P.gate_early_on && fast_warning(i)
    warn_early_t(i)=min(P.gate_early_delay,warn_early_t(i)+P.Ts);
    else
    warn_early_t(i)=0;
    end
    if spin_mask(i) || source_bad
    prewarn(i)=false; warn_armed(i)=false; warn_age(i)=0;
    warn_on_t(i)=0; warn_clear_t(i)=0; warn_early_t(i)=0;
    elseif ~prewarn(i)
    if warn_armed(i) && (warn_on_t(i)>=P.gate_warn_delay || warn_early_t(i)>=P.gate_early_delay)
    prewarn(i)=true;warn_age(i)=0;warn_clear_t(i)=0;
    warn_armed(i)=false;
    end
    else
    warn_age(i)=warn_age(i)+P.Ts;
    % Once confirmed-spin latching takes over, leave the warning
    % lane immediately; the confirmed-spin limiter owns the event.
    if dv_warning(i)<P.gate_warn_off
    warn_clear_t(i)=min(P.gate_warn_clear,warn_clear_t(i)+P.Ts);
    else
    warn_clear_t(i)=0;
    end
    if prewarn(i) && warn_age(i)>=P.gate_warn_hold && warn_clear_t(i)>=P.gate_warn_clear
    prewarn(i)=false;warn_armed(i)=true;warn_age(i)=0;warn_on_t(i)=0;warn_early_t(i)=0;
    end
    end
    end
    nspin=sum(double(spin_mask));
    if no_move_raw, no_move_t=min(P.t_no_move,no_move_t+P.Ts); elseif move_ok, no_move_t=0; else, no_move_t=max(0,no_move_t-P.Ts); end
    no_move_confirmed=no_move_t>=P.t_no_move;
    if ~speed_valid
    if speed_on_raw && nspin<=1 && ~source_bad, speed_on_t=min(P.t_speed_on,speed_on_t+P.Ts); else, speed_on_t=0; end
    if speed_on_t>=P.t_speed_on, speed_valid=true; speed_off_t=0; end
    else
    if speed_off_raw || nspin>=2 || source_bad, speed_off_t=min(P.t_speed_off,speed_off_t+P.Ts); else, speed_off_t=0; end
    if speed_off_t>=P.t_speed_off, speed_valid=false; speed_on_t=0; end
    end
    if source_bad, desired_stage=uint8(6); elseif nspin>=2, desired_stage=uint8(4);
    elseif nspin==1, desired_stage=uint8(3); elseif speed_valid, desired_stage=uint8(5);
    elseif no_move_confirmed, desired_stage=uint8(2); elseif move_ok, desired_stage=uint8(1);
    else, desired_stage=uint8(0); end
    end
    settings: executionOrder=1
  state MODE [parallel]
    settings: executionOrder=2
    state DISABLED
      entry: stage = uint8(255);
    state START_PROBE
      entry: stage = uint8(0);
    state NORMAL_LAUNCH
      entry: stage = uint8(1);
    state HEAVY_NO_MOVE
      entry: stage = uint8(2);
    state SINGLE_SPIN
      entry: stage = uint8(3);
    state MULTI_SPIN
      entry: stage = uint8(4);
    state WORK_PASS
      entry: stage = uint8(5);
    state PROTECT
      entry: stage = uint8(6);
    (default) -> DISABLED
    (junction 98) -> START_PROBE [order 2] : [desired_stage == uint8(0)]
    (junction 98) -> DISABLED [order 1] : [desired_stage == uint8(255)]
    DISABLED -> (junction 98) : [desired_stage ~= uint8(255)]
    START_PROBE -> (junction 98) : [desired_stage ~= uint8(0)]
    (junction 98) -> HEAVY_NO_MOVE [order 4] : [desired_stage == uint8(2)]
    (junction 98) -> NORMAL_LAUNCH [order 3] : [desired_stage == uint8(1)]
    HEAVY_NO_MOVE -> (junction 98) : [desired_stage ~= uint8(2)]
    NORMAL_LAUNCH -> (junction 98) : [desired_stage ~= uint8(1)]
    (junction 98) -> MULTI_SPIN [order 6] : [desired_stage == uint8(4)]
    (junction 98) -> SINGLE_SPIN [order 5] : [desired_stage == uint8(3)]
    MULTI_SPIN -> (junction 98) : [desired_stage == uint8(6) || desired_stage == uint8(255) || (desired_stage ~= uint8(4) && after(0.2,sec))]
    SINGLE_SPIN -> (junction 98) : [desired_stage == uint8(6) || desired_stage == uint8(255) || (desired_stage ~= uint8(3) && after(0.2,sec))]
    (junction 98) -> PROTECT [order 8] : [desired_stage == uint8(6)]
    PROTECT -> (junction 98) : [desired_stage ~= uint8(6)]
    (junction 98) -> WORK_PASS [order 7] : [desired_stage == uint8(5)]
    WORK_PASS -> (junction 98) : [desired_stage ~= uint8(5)]
  data: spin_on_raw input boolean size=[4 1]; spin_clear_raw input boolean size=[4 1]; no_move_raw input boolean size=1; move_ok input boolean size=1; speed_on_raw input boolean size=1; speed_off_raw input boolean size=1; consistency_ok input boolean size=1; source_immediate_bad input boolean size=1; enable input double size=1; reset input double size=1; stage output uint8; spin_mask output boolean size=[4 1]; speed_valid output boolean; no_move_confirmed output boolean; source_bad output boolean; nspin output double; P parameter; spin_on_t local size=[4 1]; spin_clear_t local size=[4 1]; no_move_t local; speed_on_t local; speed_off_t local; cons_bad_t local; desired_stage local uint8; i local double size=1; dv_warning input double size=[4 1]; fast_warning input boolean size=[4 1]; prewarn output boolean size=[4 1]; warn_age output double size=[4 1]; warn_on_t local double size=[4 1]; warn_clear_t local double size=[4 1]; warn_early_t local double size=[4 1]; warn_armed local boolean size=[4 1]
